simulink model "canal_gaussien"  (R2023b)
settings: Solver=FixedStepDiscrete  StartTime=0.0  StopTime=(N-1)*Tb  FixedStep=Tb  RelTol=1e-3
values from neighbouring files (symbols this model uses):
  A = P.A    [parametres.m]    (also in partie2_1.m; partie2_5_q10.m = numel(unique(msg)); partie2_5_q11.m = numel(unique(seq)))
  graine = P.graine    [parametres.m]    (also in parametres_perso.m = mod(sum(c .* (1:numel(c)) * 31) + 7 * numel(c), 2^31 - 1); partie2_1.m)
  p1 = P.p1    [parametres.m]    (also in partie2_1.m; partie2_4_q9.m = mean(bits))
  s = double(out.sortie(:))    [creer_codeur.m]    (also in creer_gaussien.m = sigma^2/(2*A) * log((1-p1)/p1); creer_uniforme.m = a - A; hamming_decode.m = mod(y * H', 2); parametres_perso.m = RandStream('mt19937ar', 'Seed', graine))
  sigma = P.sigma    [parametres.m]    (also in partie2_1.m)
  Tb = 1    [parametres.m]    (also in partie2_1.m)
libraries: simulink x2
settings Model: Creator=e2507477  LastModifiedBy=e2507477

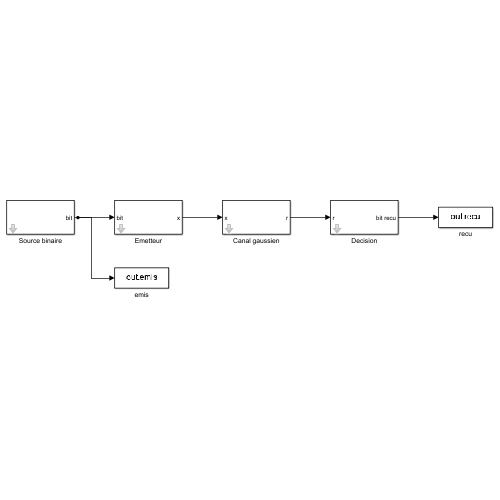
[thumbnail: Simulink's stored preview of the top-level diagram]
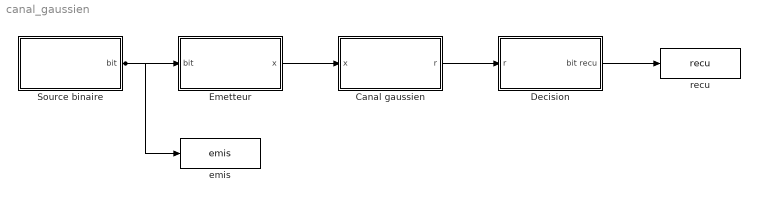
== system canal_gaussien ==
  Canal gaussien : Subsystem  mask{sigma=sigma, Tb=Tb, graine=graine}
      mask prompts: sigma "Écart-type du bruit sigma"; Tb "Durée d'un bit"
  Decision : Subsystem  mask{s=s}
      mask prompts: s "Seuil de décision s"
  Emetteur : Subsystem  mask{A=A}
      mask prompts: A "Amplitude A"
  Source binaire : Subsystem  mask{p1=p1, Tb=Tb, graine=graine}
      mask prompts: p1 "Probabilité d'un 1"; Tb "Durée d'un bit"
  emis : ToWorkspace  VariableName=emis  SampleTime=-1
  recu : ToWorkspace  VariableName=recu  SampleTime=-1
  wires:
  Source binaire/1(bit) -> Emetteur/1(bit), emis/1
  Emetteur/1(x) -> Canal gaussien/1(x)
  Canal gaussien/1(r) -> Decision/1(r)
  Decision/1(bit recu) -> recu/1

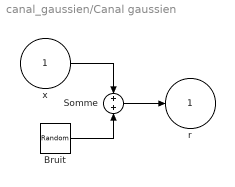
== system canal_gaussien/Canal gaussien ==
  x : Inport
  Bruit : RandomNumber  Variance=sigma^2  Seed=round(graine)+5000  SampleTime=Tb
  Somme : Sum
  r : Outport
  wires:
  x/1 -> Somme/1
  Bruit/1 -> Somme/2
  Somme/1 -> r/1

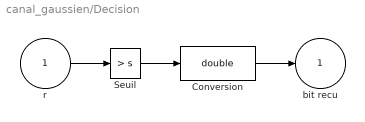
== system canal_gaussien/Decision ==
  r : Inport
  Conversion : DataTypeConversion  OutDataTypeStr=double  SaturateOnIntegerOverflow=off  RndMeth=Floor
  Seuil : simulink/Logic and Bit Operations/Compare To Constant  relop=>  const=s  OutDataTypeStr=boolean
  bit recu : Outport
  wires:
  r/1 -> Seuil/1
  Conversion/1 -> bit recu/1
  Seuil/1 -> Conversion/1

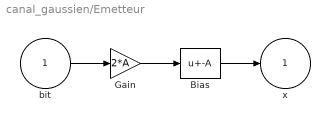
== system canal_gaussien/Emetteur ==
  bit : Inport
  Bias : Bias  Bias=-A  SaturateOnIntegerOverflow=off
  Gain : Gain  Gain=2*A
  x : Outport
  wires:
  bit/1 -> Gain/1
  Gain/1 -> Bias/1
  Bias/1 -> x/1

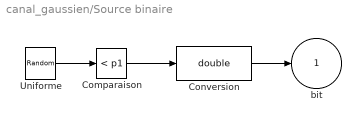
== system canal_gaussien/Source binaire ==
  Comparaison : simulink/Logic and Bit Operations/Compare To Constant  relop=<  const=p1  OutDataTypeStr=boolean
  Conversion : DataTypeConversion  OutDataTypeStr=double  SaturateOnIntegerOverflow=off  RndMeth=Floor
  Uniforme : UniformRandomNumber  Minimum=0  Seed=round(graine)  SampleTime=Tb
  bit : Outport
  wires:
  Uniforme/1 -> Comparaison/1
  Comparaison/1 -> Conversion/1
  Conversion/1 -> bit/1
